simulink model "gm_PMLSM_FOC_FixedPoint"  (R2026b)
settings: Solver=FixedStepDiscrete  StopTime=0.0063  FixedStep=2e-08
undefined symbols (not defined in the file): Lookup, Ts_ACR
libraries: hdlmdlgenlib x38, simulink x8
(part 1 of 5)
settings Model: Creator=lww  LastModifiedBy=lww
settings DataIOCC: ExternalInput=M3_HDL_Stimulus  LoadExternalInput=on
settings OptimizationCC: BlockReduction=off  ConditionallyExecuteInputs=off  DefaultParameterBehavior=Inlined
settings DebuggingCC: FixptConstOverflowMsg=error  InheritedTsInSrcMsg=none  IntegerOverflowMsg=error  IntegerSaturationMsg=error

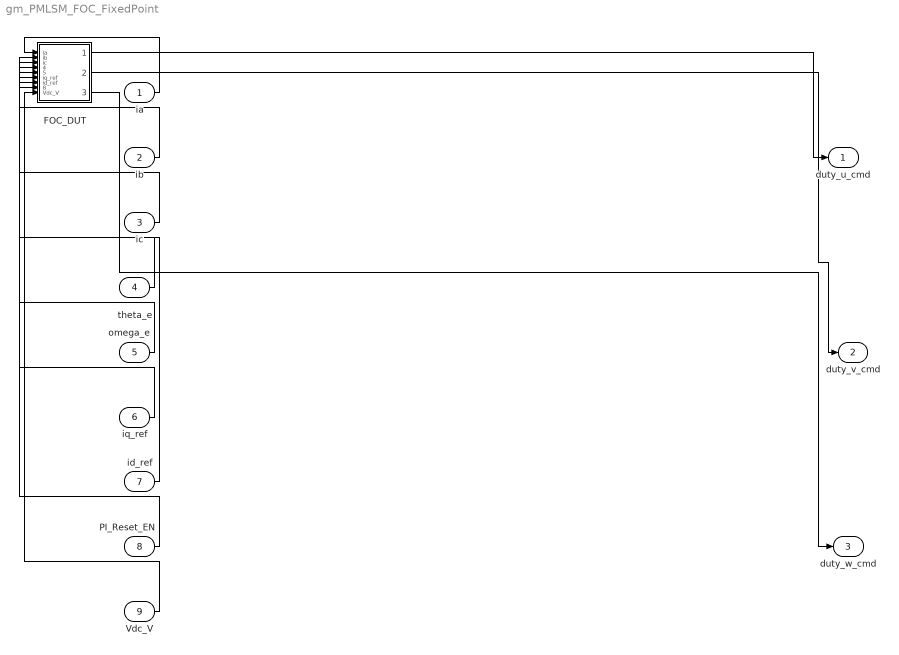
== system gm_PMLSM_FOC_FixedPoint ==
  ia : Inport  OutDataTypeStr=FOC_Fixed_Config.Types.Current  SampleTime=Ts_ACR  Interpolate=off
  ib : Inport  Port=2  OutDataTypeStr=FOC_Fixed_Config.Types.Current  SampleTime=Ts_ACR  Interpolate=off
  ic : Inport  Port=3  OutDataTypeStr=FOC_Fixed_Config.Types.Current  SampleTime=Ts_ACR  Interpolate=off
  theta_e : Inport  Port=4  OutDataTypeStr=FOC_Fixed_Config.Types.Angle  SampleTime=Ts_ACR  Interpolate=off
  omega_e : Inport  Port=5  OutDataTypeStr=FOC_Fixed_Config.Types.Omega  SampleTime=Ts_ACR  Interpolate=off
  iq_ref : Inport  Port=6  OutDataTypeStr=FOC_Fixed_Config.Types.Current  SampleTime=Ts_ACR  Interpolate=off
  id_ref : Inport  Port=7  OutDataTypeStr=FOC_Fixed_Config.Types.Current  SampleTime=Ts_ACR  Interpolate=off
  PI_Reset_EN : Inport  Port=8  OutDataTypeStr=boolean  SampleTime=Ts_ACR  Interpolate=off
  Vdc_V : Inport  Port=9  OutDataTypeStr=FOC_Fixed_Config.Types.Bus  SampleTime=Ts_ACR  Interpolate=off
  FOC_DUT : Subsystem
  duty_u_cmd : Outport  OutDataTypeStr=FOC_Fixed_Config.Types.Duty
  duty_v_cmd : Outport  Port=2  OutDataTypeStr=FOC_Fixed_Config.Types.Duty
  duty_w_cmd : Outport  Port=3  OutDataTypeStr=FOC_Fixed_Config.Types.Duty
  wires:
  Vdc_V/1 -> FOC_DUT/9(Vdc_V)
  FOC_DUT/3(duty_w_cmd) -> duty_w_cmd/1
  FOC_DUT/2(duty_v_cmd) -> duty_v_cmd/1
  FOC_DUT/1(duty_u_cmd) -> duty_u_cmd/1
  PI_Reset_EN/1 -> FOC_DUT/8(PI_Reset_EN)
  id_ref/1 -> FOC_DUT/7(id_ref)
  iq_ref/1 -> FOC_DUT/6(iq_ref)
  omega_e/1 -> FOC_DUT/5(omega_e)
  theta_e/1 -> FOC_DUT/4(theta_e)
  ic/1 -> FOC_DUT/3(ic)
  ib/1 -> FOC_DUT/2(ib)
  ia/1 -> FOC_DUT/1(ia)

== system gm_PMLSM_FOC_FixedPoint/FOC_DUT ==
  ia : Inport  OutDataTypeStr=fixdt(1, 32, 24)  PortDimensions=1  SampleTime=0.0001
  ib : Inport  Port=2  OutDataTypeStr=fixdt(1, 32, 24)  PortDimensions=1  SampleTime=0.0001
  ic : Inport  Port=3  OutDataTypeStr=fixdt(1, 32, 24)  PortDimensions=1  SampleTime=0.0001
  theta_e : Inport  Port=4  OutDataTypeStr=fixdt(1, 40, 32)  PortDimensions=1  SampleTime=0.0001
  omega_e : Inport  Port=5  OutDataTypeStr=fixdt(1, 40, 24)  PortDimensions=1  SampleTime=0.0001
  iq_ref : Inport  Port=6  OutDataTypeStr=fixdt(1, 32, 24)  PortDimensions=1  SampleTime=0.0001
  id_ref : Inport  Port=7  OutDataTypeStr=fixdt(1, 32, 24)  PortDimensions=1  SampleTime=0.0001
  PI_Reset_EN : Inport  Port=8  OutDataTypeStr=boolean  PortDimensions=1  SampleTime=0.0001
  Vdc_V : Inport  Port=9  OutDataTypeStr=fixdt(0, 32, 24)  PortDimensions=1  SampleTime=0.0001
  FOC_DUT : Subsystem  TreatAsAtomicUnit=on
  t : RateTransition  OutPortSampleTimeOpt=Multiple of input port sample time  OutPortSampleTimeMultiple=5000
  t1 : RateTransition  OutPortSampleTimeOpt=Multiple of input port sample time  OutPortSampleTimeMultiple=5000
  t2 : RateTransition  OutPortSampleTimeOpt=Multiple of input port sample time  OutPortSampleTimeMultiple=5000
  duty_u_cmd : Outport  OutDataTypeStr=fixdt(0, 32, 30)  PortDimensions=1  SampleTime=0.0001
  duty_v_cmd : Outport  Port=2  OutDataTypeStr=fixdt(0, 32, 30)  PortDimensions=1  SampleTime=0.0001
  duty_w_cmd : Outport  Port=3  OutDataTypeStr=fixdt(0, 32, 30)  PortDimensions=1  SampleTime=0.0001
  wires:
  id_ref/1 -> FOC_DUT/7(id_ref)
  iq_ref/1 -> FOC_DUT/6(iq_ref)
  omega_e/1 -> FOC_DUT/5(omega_e)
  theta_e/1 -> FOC_DUT/4(theta_e)
  ic/1 -> FOC_DUT/3(ic)
  ia/1 -> FOC_DUT/1(ia)
  ib/1 -> FOC_DUT/2(ib)
  PI_Reset_EN/1 -> FOC_DUT/8(PI_Reset_EN)
  FOC_DUT/2(duty_v_cmd) -> t1/1
  Vdc_V/1 -> FOC_DUT/9(Vdc_V)
  FOC_DUT/1(duty_u_cmd) -> t/1
  FOC_DUT/3(duty_w_cmd) -> t2/1
  t/1 -> duty_u_cmd/1
  t1/1 -> duty_v_cmd/1
  t2/1 -> duty_w_cmd/1

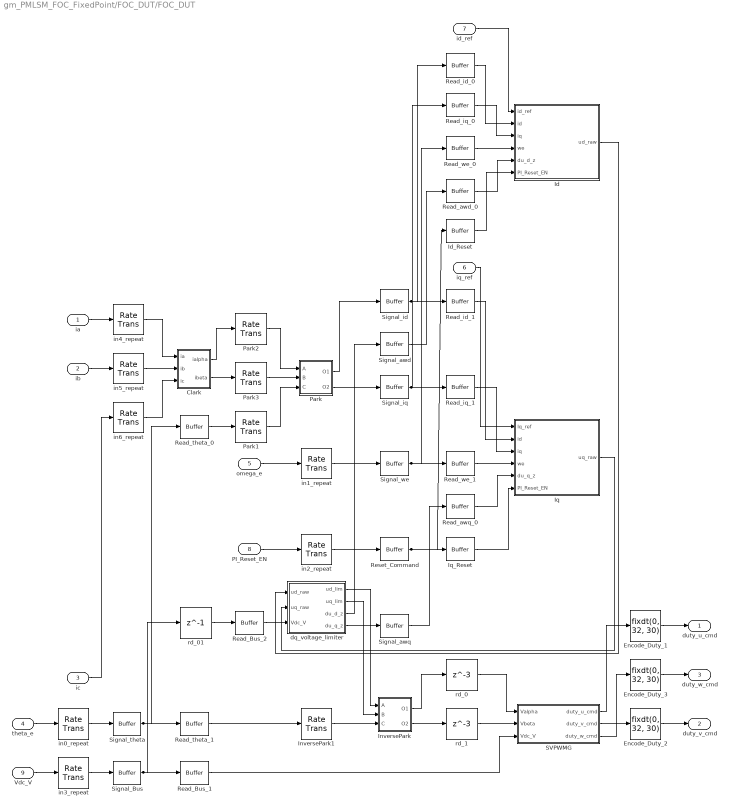
== system gm_PMLSM_FOC_FixedPoint/FOC_DUT/FOC_DUT ==
  ia : Inport  OutDataTypeStr=fixdt(1,32,24,'DataTypeOverride', 'Off')  PortDimensions=1  SampleTime=0.0001
  ib : Inport  Port=2  OutDataTypeStr=fixdt(1,32,24,'DataTypeOverride', 'Off')  PortDimensions=1  SampleTime=0.0001
  ic : Inport  Port=3  OutDataTypeStr=fixdt(1,32,24,'DataTypeOverride', 'Off')  PortDimensions=1  SampleTime=0.0001
  theta_e : Inport  Port=4  OutDataTypeStr=fixdt(1,40,32,'DataTypeOverride', 'Off')  PortDimensions=1  SampleTime=0.0001
  omega_e : Inport  Port=5  OutDataTypeStr=fixdt(1,40,24,'DataTypeOverride', 'Off')  PortDimensions=1  SampleTime=0.0001
  iq_ref : Inport  Port=6  OutDataTypeStr=fixdt(1,32,24,'DataTypeOverride', 'Off')  PortDimensions=1  SampleTime=0.0001
  id_ref : Inport  Port=7  OutDataTypeStr=fixdt(1,32,24,'DataTypeOverride', 'Off')  PortDimensions=1  SampleTime=0.0001
  PI_Reset_EN : Inport  Port=8  OutDataTypeStr=boolean  PortDimensions=1  SampleTime=0.0001
  Vdc_V : Inport  Port=9  OutDataTypeStr=fixdt(0,32,24,'DataTypeOverride', 'Off')  PortDimensions=1  SampleTime=0.0001
  Clark : Subsystem
  Encode_Duty_1 : DataTypeConversion  OutDataTypeStr=fixdt(0, 32, 30)  RndMeth=Convergent  SampleTime=2e-08
  Encode_Duty_2 : DataTypeConversion  OutDataTypeStr=fixdt(0, 32, 30)  RndMeth=Convergent  SampleTime=2e-08
  Encode_Duty_3 : DataTypeConversion  OutDataTypeStr=fixdt(0, 32, 30)  RndMeth=Convergent  SampleTime=2e-08
  Id : Subsystem
  Id_Reset : hdlmdlgenlib/Buffer
  InversePark : Subsystem  mask(Park to Clarke Angle Transform){AxisAlignment=D-axis, UseWithEmbedded=on, PhaseInput='Two inputs', ThetaInput=Electrical position, AngleInput=Radians, N_points=1024}
      mask prompts: AxisAlignment "shared_mcbeeblks:mcbeeblks:InvPBlkPrmAlign"; UseWithEmbedded "shared_mcbeeblks:mcbeeblks:BlkEmbeddedUse"; PhaseInput "shared_mcbeeblks:mcbeeblks:InvPPrmInp"; ThetaInput "shared_mcbeeblks:mcbeeblks:InvPPrmTheta"; AngleInput "shared_mcbeeblks:mcbeeblks:InvPThetaUnits"; N_points "shared_mcbeeblks:mcbeeblks:InvPPrmLUTSize"
      mask help: shared_mcbeeblks:mcbeeblks:InvPBlkDlgDes
      mask init:
      | AngleInput = 2;
      | AxisAlignment = 1;
      | N_points = 1024;
      | PhaseInput = 1;
      | ThetaInput = 1;
      | UseWithEmbedded = 1;
      mask Help: eval('mcbeeutil.mcbeesharedhelp(''inverseparktransform'')')
      mask TypeOptions AxisAlignment: shared_mcbeeblks:mcbeeblks:InvPpopDaxis | shared_mcbeeblks:mcbeeblks:InvPpopQaxis
      mask Callback UseWithEmbedded: mcbeeutil.mcbeeParkToClarkeCb('embeddeduse',gcbh);
      mask TypeOptions ThetaInput: shared_mcbeeblks:mcbeeblks:InvPPopElec | shared_mcbeeblks:mcbeeblks:InvPPopSinCos
      mask Callback ThetaInput: mcbeeutil.mcbeeParkToClarkeCb('ThetaInputCb',gcbh);
      mask TypeOptions AngleInput: shared_mcbeeblks:mcbeeblks:InvPPopPUUnit | shared_mcbeeblks:mcbeeblks:InvPPopRadUnit | shared_mcbeeblks:mcbeeblks:InvPPopDegUnit
      mask Display:
      | fprintf('Park to\nClarke')
      | port_label('input',1, 'd','interpreter', 'tex');
      | port_label('input',2, 'q','interpreter', 'tex');
      | port_label('input',3, '\theta_e','interpreter', 'tex');
      | port_label('output',1, '\alpha','interpreter', 'tex');
      | port_label('output',2, '\beta','interpreter', 'tex');
  InversePark1 : RateTransition  OutPortSampleTimeOpt=Multiple of input port sample time  OutPortSampleTimeMultiple=5000
  Iq : Subsystem
  Iq_Reset : hdlmdlgenlib/Buffer
  Park : Subsystem  mask(Clarke to Park Angle Transform){AxisAlignment=D-axis, UseWithEmbedded=on, PhaseInput='Two inputs', ThetaInput=Electrical position, AngleInput=Radians, N_points=1024}
      mask prompts: AxisAlignment "shared_mcbeeblks:mcbeeblks:ParkBlkPrmAlign"; UseWithEmbedded "shared_mcbeeblks:mcbeeblks:BlkEmbeddedUse"; PhaseInput "shared_mcbeeblks:mcbeeblks:ParkPrmInp"; ThetaInput "shared_mcbeeblks:mcbeeblks:ParkPrmTheta"; AngleInput "shared_mcbeeblks:mcbeeblks:ParkPrmThetaUnits"; N_points "shared_mcbeeblks:mcbeeblks:ParkPrmLUTSize"
      mask help: shared_mcbeeblks:mcbeeblks:ParkBlkDlgDes
      mask init:
      | AngleInput = 2;
      | AxisAlignment = 1;
      | N_points = 1024;
      | PhaseInput = 1;
      | ThetaInput = 1;
      | UseWithEmbedded = 1;
      mask Help: eval('mcbeeutil.mcbeesharedhelp(''parktransform'')')
      mask TypeOptions AxisAlignment: shared_mcbeeblks:mcbeeblks:ParkpopDaxis | shared_mcbeeblks:mcbeeblks:ParkpopQaxis
      mask Callback UseWithEmbedded: mcbeeutil.mcbeeClarkeToParkCb('embeddeduse',gcbh);
      mask TypeOptions ThetaInput: shared_mcbeeblks:mcbeeblks:ParkPopElec | shared_mcbeeblks:mcbeeblks:ParkPopSinCos
      mask Callback ThetaInput: mcbeeutil.mcbeeClarkeToParkCb('ThetaInputCb',gcbh)
      mask TypeOptions AngleInput: shared_mcbeeblks:mcbeeblks:ParkPopPUUnit | shared_mcbeeblks:mcbeeblks:ParkPopRadUnit | shared_mcbeeblks:mcbeeblks:ParkPopDegUnit
      mask Display:
      | fprintf('Clarke to\nPark')
      | port_label('input',1, '\alpha','interpreter', 'tex');
      | port_label('input',2, '\beta','interpreter', 'tex');
      | port_label('input',3, '\theta_e','interpreter', 'tex');
      | port_label('output',1, 'd','interpreter', 'tex');
      | port_label('output',2, 'q','interpreter', 'tex');
  Park1 : RateTransition  OutPortSampleTimeOpt=Multiple of input port sample time  OutPortSampleTimeMultiple=5000
  Park2 : RateTransition  OutPortSampleTimeOpt=Multiple of input port sample time  OutPortSampleTimeMultiple=5000
  Park3 : RateTransition  OutPortSampleTimeOpt=Multiple of input port sample time  OutPortSampleTimeMultiple=5000
  Read_Bus_1 : hdlmdlgenlib/Buffer
  Read_Bus_2 : hdlmdlgenlib/Buffer
  Read_awd_0 : hdlmdlgenlib/Buffer
  Read_awq_0 : hdlmdlgenlib/Buffer
  Read_id_0 : hdlmdlgenlib/Buffer
  Read_id_1 : hdlmdlgenlib/Buffer
  Read_iq_0 : hdlmdlgenlib/Buffer
  Read_iq_1 : hdlmdlgenlib/Buffer
  Read_theta_0 : hdlmdlgenlib/Buffer
  Read_theta_1 : hdlmdlgenlib/Buffer
  Read_we_0 : hdlmdlgenlib/Buffer
  Read_we_1 : hdlmdlgenlib/Buffer
  Reset_Command : hdlmdlgenlib/Buffer
  SVPWMG : Subsystem
  Signal_Bus : hdlmdlgenlib/Buffer
  Signal_awd : hdlmdlgenlib/Buffer
  Signal_awq : hdlmdlgenlib/Buffer
  Signal_id : hdlmdlgenlib/Buffer
  Signal_iq : hdlmdlgenlib/Buffer
  Signal_theta : hdlmdlgenlib/Buffer
  Signal_we : hdlmdlgenlib/Buffer
  dq_voltage_limiter : Subsystem
  in0_repeat : RateTransition  Integrity=off  Deterministic=off  OutPortSampleTimeOpt=Multiple of input port sample time  OutPortSampleTimeMultiple=1/5000
  in1_repeat : RateTransition  Integrity=off  Deterministic=off  OutPortSampleTimeOpt=Multiple of input port sample time  OutPortSampleTimeMultiple=1/5000
  in2_repeat : RateTransition  Integrity=off  Deterministic=off  OutPortSampleTimeOpt=Multiple of input port sample time  OutPortSampleTimeMultiple=1/5000
  in3_repeat : RateTransition  Integrity=off  Deterministic=off  OutPortSampleTimeOpt=Multiple of input port sample time  OutPortSampleTimeMultiple=1/5000
  in4_repeat : RateTransition  Integrity=off  Deterministic=off  OutPortSampleTimeOpt=Multiple of input port sample time  OutPortSampleTimeMultiple=1/5000
  in5_repeat : RateTransition  Integrity=off  Deterministic=off  OutPortSampleTimeOpt=Multiple of input port sample time  OutPortSampleTimeMultiple=1/5000
  in6_repeat : RateTransition  Integrity=off  Deterministic=off  OutPortSampleTimeOpt=Multiple of input port sample time  OutPortSampleTimeMultiple=1/5000
  rd_0 : Delay  DelayLength=3  InitialCondition=0  SampleTime=2e-08
  rd_01 : Delay  DelayLength=1  InitialCondition=0  SampleTime=2e-08
  rd_1 : Delay  DelayLength=3  InitialCondition=0  SampleTime=2e-08
  duty_u_cmd : Outport  OutDataTypeStr=fixdt(0,32,30,'DataTypeOverride', 'Off')  PortDimensions=1  SampleTime=2e-08
  duty_v_cmd : Outport  Port=2  OutDataTypeStr=fixdt(0,32,30,'DataTypeOverride', 'Off')  PortDimensions=1  SampleTime=2e-08
  duty_w_cmd : Outport  Port=3  OutDataTypeStr=fixdt(0,32,30,'DataTypeOverride', 'Off')  PortDimensions=1  SampleTime=2e-08
  wires:
  Signal_id/1 -> Read_id_1/1, Read_id_0/1
  theta_e/1 -> in0_repeat/1
  ia/1 -> in4_repeat/1
  Vdc_V/1 -> in3_repeat/1
  in3_repeat/1 -> Signal_Bus/1
  ib/1 -> in5_repeat/1
  SVPWMG/3(duty_w_cmd) -> Encode_Duty_3/1
  Signal_Bus/1 -> Read_Bus_1/1, rd_01/1
  ic/1 -> in6_repeat/1
  Read_awd_0/1 -> Id/5(du_d_z)
  in0_repeat/1 -> Signal_theta/1
  dq_voltage_limiter/2(uq_lim) -> InversePark/2(B)
  in4_repeat/1 -> Clark/1(ia)
  in5_repeat/1 -> Clark/2(ib)
  rd_1/1 -> SVPWMG/2(Vbeta)
  Reset_Command/1 -> Iq_Reset/1, Id_Reset/1
  in6_repeat/1 -> Clark/3(ic)
  Signal_theta/1 -> Read_theta_0/1, Read_theta_1/1
  Clark/1(ialpha) -> Park2/1
  Read_id_0/1 -> Id/2(id)
  Clark/2(ibeta) -> Park3/1
  InversePark/2(O2) -> rd_1/1
  Read_theta_0/1 -> Park1/1
  Encode_Duty_2/1 -> duty_v_cmd/1
  Signal_awq/1 -> Read_awq_0/1
  rd_01/1 -> Read_Bus_2/1
  Read_theta_1/1 -> InversePark1/1
  Read_Bus_1/1 -> SVPWMG/3(Vdc_V)
  Id/1(ud_raw) -> dq_voltage_limiter/1(ud_raw)
  Iq_Reset/1 -> Iq/6(PI_Reset_EN)
  Park2/1 -> Park/1(A)
  Park3/1 -> Park/2(B)
  Park1/1 -> Park/3(C)
  omega_e/1 -> in1_repeat/1
  PI_Reset_EN/1 -> in2_repeat/1
  id_ref/1 -> Id/1(id_ref)
  Read_Bus_2/1 -> dq_voltage_limiter/3(Vdc_V)
  Park/1(O1) -> Signal_id/1
  SVPWMG/2(duty_v_cmd) -> Encode_Duty_2/1
  Park/2(O2) -> Signal_iq/1
  Id_Reset/1 -> Id/6(PI_Reset_EN)
  in1_repeat/1 -> Signal_we/1
  in2_repeat/1 -> Reset_Command/1
  Encode_Duty_1/1 -> duty_u_cmd/1
  dq_voltage_limiter/1(ud_lim) -> InversePark/1(A)
  Read_we_1/1 -> Iq/4(we)
  dq_voltage_limiter/3(du_d_z) -> Signal_awd/1
  SVPWMG/1(duty_u_cmd) -> Encode_Duty_1/1
  dq_voltage_limiter/4(du_q_z) -> Signal_awq/1
  InversePark1/1 -> InversePark/3(C)
  Signal_awd/1 -> Read_awd_0/1
  Signal_iq/1 -> Read_iq_1/1, Read_iq_0/1
  Signal_we/1 -> Read_we_1/1, Read_we_0/1
  InversePark/1(O1) -> rd_0/1
  Read_iq_0/1 -> Id/3(iq)
  Read_we_0/1 -> Id/4(we)
  iq_ref/1 -> Iq/1(Iq_ref)
  rd_0/1 -> SVPWMG/1(Valpha)
  Read_id_1/1 -> Iq/2(id)
  Read_iq_1/1 -> Iq/3(iq)
  Read_awq_0/1 -> Iq/5(du_q_z)
  Iq/1(uq_raw) -> dq_voltage_limiter/2(uq_raw)
  Encode_Duty_3/1 -> duty_w_cmd/1

== system gm_PMLSM_FOC_FixedPoint/FOC_DUT/FOC_DUT/Clark ==
  ia : Inport  OutDataTypeStr=fixdt(1, 32, 24)  PortDimensions=1  SampleTime=2e-08
  ib : Inport  Port=2  OutDataTypeStr=fixdt(1, 32, 24)  PortDimensions=1  SampleTime=2e-08
  ic : Inport  Port=3  OutDataTypeStr=fixdt(1, 32, 24)  PortDimensions=1  SampleTime=2e-08
  Add1 : Sum  Inputs=+-  OutDataTypeStr=fixdt(1, 64, 40)  AccumDataTypeStr=fixdt(1, 64, 40)  RndMeth=Convergent  SaturateOnIntegerOverflow=on  SampleTime=2e-08
  Add_stage2 : Sum  Inputs=+-  OutDataTypeStr=fixdt(1, 64, 40)  AccumDataTypeStr=fixdt(1, 64, 40)  RndMeth=Convergent  SaturateOnIntegerOverflow=on  SampleTime=2e-08
  Add_stage3 : Sum  Inputs=+-  OutDataTypeStr=fixdt(1, 64, 40)  AccumDataTypeStr=fixdt(1, 64, 40)  RndMeth=Convergent  SaturateOnIntegerOverflow=on  SampleTime=2e-08
  Gain : Gain  Gain="fi(0,1,64,40,\"hex\",\"0000008000000000\")"  ParamDataTypeStr=fixdt(1, 64, 40)  OutDataTypeStr=fixdt(1, 64, 40)  RndMeth=Convergent  SaturateOnIntegerOverflow=on  SampleTime=2e-08
  Gain1 : Gain  Gain="fi(0,1,64,40,\"hex\",\"0000008000000000\")"  ParamDataTypeStr=fixdt(1, 64, 40)  OutDataTypeStr=fixdt(1, 64, 40)  RndMeth=Convergent  SaturateOnIntegerOverflow=on  SampleTime=2e-08
  Gain2 : Gain  Gain="fi(0,1,64,40,\"hex\",\"000000aaaaaaaaab\")"  ParamDataTypeStr=fixdt(1, 64, 40)  OutDataTypeStr=fixdt(1, 128, 80)  SampleTime=2e-08
  Gain2_out_dtc : DataTypeConversion  OutDataTypeStr=fixdt(1, 64, 40)  RndMeth=Convergent  SampleTime=2e-08
  Gain3 : Gain  Gain="fi(0,1,64,40,\"hex\",\"00000093cd3a2c82\")"  ParamDataTypeStr=fixdt(1, 64, 40)  OutDataTypeStr=fixdt(1, 128, 80)  SampleTime=2e-08
  Gain3_out_dtc : DataTypeConversion  OutDataTypeStr=fixdt(1, 64, 40)  RndMeth=Convergent  SampleTime=2e-08
  ialpha : Outport  OutDataTypeStr=fixdt(1, 64, 40)  PortDimensions=1  SampleTime=2e-08
  ibeta : Outport  Port=2  OutDataTypeStr=fixdt(1, 64, 40)  PortDimensions=1  SampleTime=2e-08
  wires:
  Gain1/1 -> Add_stage3/2
  ib/1 -> Add1/1, Gain/1
  Add1/1 -> Gain3/1
  ic/1 -> Gain1/1, Add1/2
  Gain/1 -> Add_stage2/2
  ia/1 -> Add_stage2/1
  Add_stage2/1 -> Add_stage3/1
  Gain3/1 -> Gain3_out_dtc/1
  Add_stage3/1 -> Gain2/1
  Gain3_out_dtc/1 -> ibeta/1
  Gain2/1 -> Gain2_out_dtc/1
  Gain2_out_dtc/1 -> ialpha/1

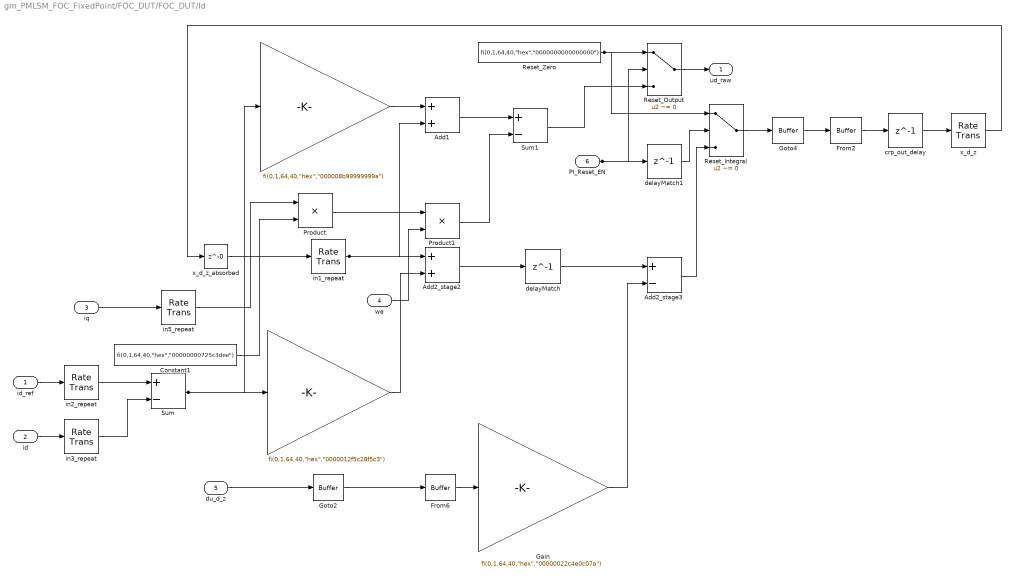
== system gm_PMLSM_FOC_FixedPoint/FOC_DUT/FOC_DUT/Id ==
  id_ref : Inport  OutDataTypeStr=fixdt(1, 32, 24)  PortDimensions=1  SampleTime=0.0001
  id : Inport  Port=2  OutDataTypeStr=fixdt(1, 64, 40)  PortDimensions=1  SampleTime=0.0001
  iq : Inport  Port=3  OutDataTypeStr=fixdt(1, 64, 40)  PortDimensions=1  SampleTime=0.0001
  we : Inport  Port=4  OutDataTypeStr=fixdt(1, 40, 24)  PortDimensions=1  SampleTime=2e-08
  du_d_z : Inport  Port=5  OutDataTypeStr=fixdt(1, 64, 40)  PortDimensions=1  SampleTime=2e-08
  PI_Reset_EN : Inport  Port=6  OutDataTypeStr=boolean  PortDimensions=1  SampleTime=2e-08
  " " : Gain  Gain="fi(0,1,64,40,\"hex\",\"0000012f5c28f5c3\")"  ParamDataTypeStr=fixdt(1, 64, 40)  OutDataTypeStr=fixdt(1, 64, 40)  RndMeth=Convergent  SaturateOnIntegerOverflow=on  SampleTime=2e-08
  "  " : Gain  Gain="fi(0,1,64,40,\"hex\",\"000008b99999999a\")"  ParamDataTypeStr=fixdt(1, 64, 40)  OutDataTypeStr=fixdt(1, 64, 40)  RndMeth=Convergent  SaturateOnIntegerOverflow=on  SampleTime=2e-08
  Add1 : Sum  OutDataTypeStr=fixdt(1, 64, 40)  AccumDataTypeStr=fixdt(1, 64, 40)  RndMeth=Convergent  SaturateOnIntegerOverflow=on  SampleTime=2e-08
  Add2_stage2 : Sum  OutDataTypeStr=fixdt(1, 64, 40)  AccumDataTypeStr=fixdt(1, 64, 40)  RndMeth=Convergent  SaturateOnIntegerOverflow=on  SampleTime=2e-08
  Add2_stage3 : Sum  Inputs=+-  OutDataTypeStr=fixdt(1, 64, 40)  AccumDataTypeStr=fixdt(1, 64, 40)  RndMeth=Convergent  SaturateOnIntegerOverflow=on  SampleTime=2e-08
  Constant1 : Constant  Value="fi(0,1,64,40,\"hex\",\"00000000725c3dee\")"  OutDataTypeStr=fixdt(1, 64, 40)  SampleTime=2e-08
  From2 : hdlmdlgenlib/Buffer
  From6 : hdlmdlgenlib/Buffer
  Gain : Gain  Gain="fi(0,1,64,40,\"hex\",\"00000022c4e0c07a\")"  ParamDataTypeStr=fixdt(1, 64, 40)  OutDataTypeStr=fixdt(1, 64, 40)  RndMeth=Convergent  SaturateOnIntegerOverflow=on  SampleTime=2e-08
  Goto2 : hdlmdlgenlib/Buffer
  Goto4 : hdlmdlgenlib/Buffer
  Product : Product  Inputs=**  OutDataTypeStr=fixdt(1, 64, 40)  RndMeth=Convergent  SaturateOnIntegerOverflow=on  SampleTime=2e-08
  Product1 : Product  Inputs=**  OutDataTypeStr=fixdt(1, 64, 40)  RndMeth=Convergent  SaturateOnIntegerOverflow=on  SampleTime=2e-08
  Reset_Integral : Switch  Criteria=u2 ~= 0  Threshold="fi(0,0,1,0,\"hex\",\"0\")"  OutDataTypeStr=fixdt(1, 64, 40)  RndMeth=Convergent  SampleTime=2e-08  InputSameDT=off
  Reset_Output : Switch  Criteria=u2 ~= 0  Threshold="fi(0,0,1,0,\"hex\",\"0\")"  OutDataTypeStr=fixdt(1, 64, 40)  RndMeth=Convergent  SampleTime=2e-08  InputSameDT=off
  Reset_Zero : Constant  Value="fi(0,1,64,40,\"hex\",\"0000000000000000\")"  OutDataTypeStr=fixdt(1, 64, 40)  SampleTime=2e-08
  Sum : Sum  Inputs=+-  OutDataTypeStr=fixdt(1, 64, 40)  AccumDataTypeStr=fixdt(1, 64, 40)  RndMeth=Convergent  SaturateOnIntegerOverflow=on  SampleTime=2e-08
  Sum1 : Sum  Inputs=+-  OutDataTypeStr=fixdt(1, 64, 40)  AccumDataTypeStr=fixdt(1, 64, 40)  RndMeth=Convergent  SaturateOnIntegerOverflow=on  SampleTime=2e-08
  crp_out_delay : Delay  DelayLength=1  InitialCondition=0  SampleTime=2e-08
  delayMatch : Delay  DelayLength=1  InitialCondition=0  SampleTime=2e-08
  delayMatch1 : Delay  DelayLength=1  InitialCondition=0  SampleTime=2e-08
  in1_repeat : RateTransition  Integrity=off  Deterministic=off  OutPortSampleTimeOpt=Multiple of input port sample time  OutPortSampleTimeMultiple=1/5000
  in2_repeat : RateTransition  Integrity=off  Deterministic=off  OutPortSampleTimeOpt=Multiple of input port sample time  OutPortSampleTimeMultiple=1/5000
  in3_repeat : RateTransition  Integrity=off  Deterministic=off  OutPortSampleTimeOpt=Multiple of input port sample time  OutPortSampleTimeMultiple=1/5000
  in5_repeat : RateTransition  Integrity=off  Deterministic=off  OutPortSampleTimeOpt=Multiple of input port sample time  OutPortSampleTimeMultiple=1/5000
  x_d_z : RateTransition  OutPortSampleTimeOpt=Multiple of input port sample time  OutPortSampleTimeMultiple=5000
  x_d_z_absorbed : Delay  DelayLength=0
  ud_raw : Outport  OutDataTypeStr=fixdt(1, 64, 40)  PortDimensions=1  SampleTime=2e-08
  wires:
  From6/1 -> Gain/1
  Goto2/1 -> From6/1
  in5_repeat/1 -> Product/1
  id_ref/1 -> in2_repeat/1
  x_d_z_absorbed/1 -> in1_repeat/1
  id/1 -> in3_repeat/1
  in3_repeat/1 -> Sum/2
  iq/1 -> in5_repeat/1
  in2_repeat/1 -> Sum/1
  Constant1/1 -> Product/2
  we/1 -> Product1/2
  Sum/1 -> "  "/1, " "/1
  Product1/1 -> Sum1/2
  du_d_z/1 -> Goto2/1
  "  "/1 -> Add1/1
  Product/1 -> Product1/1
  in1_repeat/1 -> Add1/2, Add2_stage2/1
  " "/1 -> Add2_stage2/2
  Add1/1 -> Sum1/1
  Add2_stage2/1 -> delayMatch/1
  PI_Reset_EN/1 -> delayMatch1/1, Reset_Output/2
  Reset_Zero/1 -> Reset_Integral/1, Reset_Output/1
  Sum1/1 -> Reset_Output/3
  delayMatch/1 -> Add2_stage3/1
  x_d_z/1 -> x_d_z_absorbed/1
  Gain/1 -> Add2_stage3/2
  Reset_Output/1 -> ud_raw/1
  delayMatch1/1 -> Reset_Integral/2
  Add2_stage3/1 -> Reset_Integral/3
  Reset_Integral/1 -> Goto4/1
  Goto4/1 -> From2/1
  From2/1 -> crp_out_delay/1
  crp_out_delay/1 -> x_d_z/1

== system gm_PMLSM_FOC_FixedPoint/FOC_DUT/FOC_DUT/InversePark ==
  A : Inport  OutDataTypeStr=fixdt(1,64,40,'DataTypeOverride', 'Off')  PortDimensions=1  SampleTime=2e-08
  B : Inport  Port=2  OutDataTypeStr=fixdt(1,64,40,'DataTypeOverride', 'Off')  PortDimensions=1  SampleTime=2e-08
  C : Inport  Port=3  OutDataTypeStr=fixdt(1,40,32,'DataTypeOverride', 'Off')  PortDimensions=1  SampleTime=0.0001
  Variant : Subsystem
  O1 : Outport  OutDataTypeStr=fixdt(1, 64, 40)  PortDimensions=1  SampleTime=2e-08
  O2 : Outport  Port=2  OutDataTypeStr=fixdt(1, 64, 40)  PortDimensions=1  SampleTime=2e-08
  wires:
  A/1 -> Variant/1(A)
  B/1 -> Variant/2(B)
  C/1 -> Variant/3(C)
  Variant/1(O1) -> O1/1
  Variant/2(O2) -> O2/1

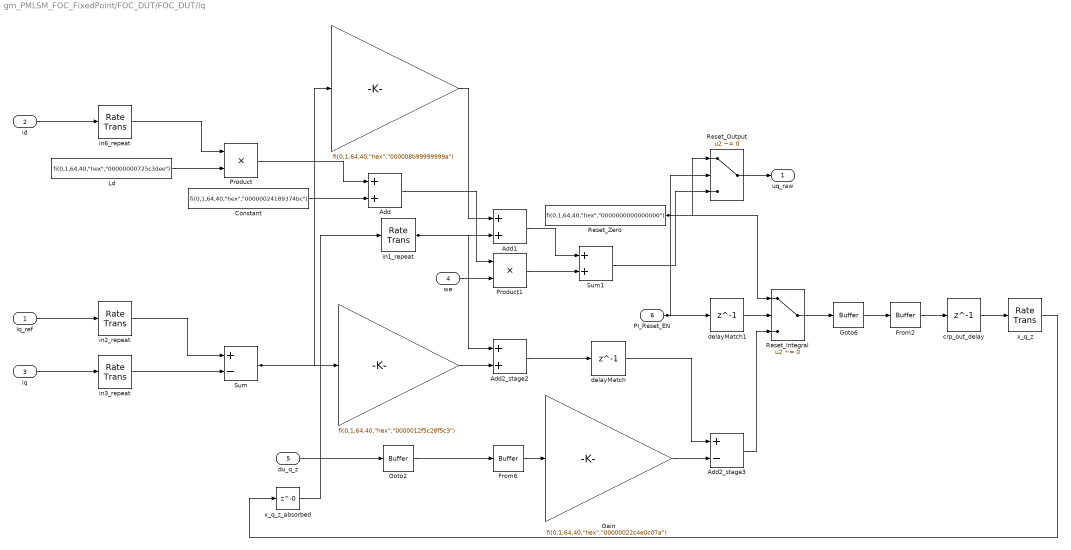
== system gm_PMLSM_FOC_FixedPoint/FOC_DUT/FOC_DUT/Iq ==
  Iq_ref : Inport  OutDataTypeStr=fixdt(1, 32, 24)  PortDimensions=1  SampleTime=0.0001
  id : Inport  Port=2  OutDataTypeStr=fixdt(1, 64, 40)  PortDimensions=1  SampleTime=0.0001
  iq : Inport  Port=3  OutDataTypeStr=fixdt(1, 64, 40)  PortDimensions=1  SampleTime=0.0001
  we : Inport  Port=4  OutDataTypeStr=fixdt(1, 40, 24)  PortDimensions=1  SampleTime=2e-08
  du_q_z : Inport  Port=5  OutDataTypeStr=fixdt(1, 64, 40)  PortDimensions=1  SampleTime=2e-08
  PI_Reset_EN : Inport  Port=6  OutDataTypeStr=boolean  PortDimensions=1  SampleTime=2e-08
  " " : Gain  Gain="fi(0,1,64,40,\"hex\",\"0000012f5c28f5c3\")"  ParamDataTypeStr=fixdt(1, 64, 40)  OutDataTypeStr=fixdt(1, 64, 40)  RndMeth=Convergent  SaturateOnIntegerOverflow=on  SampleTime=2e-08
  "  " : Gain  Gain="fi(0,1,64,40,\"hex\",\"000008b99999999a\")"  ParamDataTypeStr=fixdt(1, 64, 40)  OutDataTypeStr=fixdt(1, 64, 40)  RndMeth=Convergent  SaturateOnIntegerOverflow=on  SampleTime=2e-08
  Add : Sum  OutDataTypeStr=fixdt(1, 64, 40)  AccumDataTypeStr=fixdt(1, 64, 40)  RndMeth=Convergent  SaturateOnIntegerOverflow=on  SampleTime=2e-08
  Add1 : Sum  OutDataTypeStr=fixdt(1, 64, 40)  AccumDataTypeStr=fixdt(1, 64, 40)  RndMeth=Convergent  SaturateOnIntegerOverflow=on  SampleTime=2e-08
  Add2_stage2 : Sum  OutDataTypeStr=fixdt(1, 64, 40)  AccumDataTypeStr=fixdt(1, 64, 40)  RndMeth=Convergent  SaturateOnIntegerOverflow=on  SampleTime=2e-08
  Add2_stage3 : Sum  Inputs=+-  OutDataTypeStr=fixdt(1, 64, 40)  AccumDataTypeStr=fixdt(1, 64, 40)  RndMeth=Convergent  SaturateOnIntegerOverflow=on  SampleTime=2e-08
  Constant : Constant  Value="fi(0,1,64,40,\"hex\",\"00000024189374bc\")"  OutDataTypeStr=fixdt(1, 64, 40)  SampleTime=2e-08
  From2 : hdlmdlgenlib/Buffer
  From6 : hdlmdlgenlib/Buffer
  Gain : Gain  Gain="fi(0,1,64,40,\"hex\",\"00000022c4e0c07a\")"  ParamDataTypeStr=fixdt(1, 64, 40)  OutDataTypeStr=fixdt(1, 64, 40)  RndMeth=Convergent  SaturateOnIntegerOverflow=on  SampleTime=2e-08
  Goto2 : hdlmdlgenlib/Buffer
  Goto6 : hdlmdlgenlib/Buffer
  Ld : Constant  Value="fi(0,1,64,40,\"hex\",\"00000000725c3dee\")"  OutDataTypeStr=fixdt(1, 64, 40)  SampleTime=2e-08
  Product : Product  Inputs=**  OutDataTypeStr=fixdt(1, 64, 40)  RndMeth=Convergent  SaturateOnIntegerOverflow=on  SampleTime=2e-08
  Product1 : Product  Inputs=**  OutDataTypeStr=fixdt(1, 64, 40)  RndMeth=Convergent  SaturateOnIntegerOverflow=on  SampleTime=2e-08
  Reset_Integral : Switch  Criteria=u2 ~= 0  Threshold="fi(0,0,1,0,\"hex\",\"0\")"  OutDataTypeStr=fixdt(1, 64, 40)  RndMeth=Convergent  SampleTime=2e-08  InputSameDT=off
  Reset_Output : Switch  Criteria=u2 ~= 0  Threshold="fi(0,0,1,0,\"hex\",\"0\")"  OutDataTypeStr=fixdt(1, 64, 40)  RndMeth=Convergent  SampleTime=2e-08  InputSameDT=off
  Reset_Zero : Constant  Value="fi(0,1,64,40,\"hex\",\"0000000000000000\")"  OutDataTypeStr=fixdt(1, 64, 40)  SampleTime=2e-08
  Sum : Sum  Inputs=+-  OutDataTypeStr=fixdt(1, 64, 40)  AccumDataTypeStr=fixdt(1, 64, 40)  RndMeth=Convergent  SaturateOnIntegerOverflow=on  SampleTime=2e-08
  Sum1 : Sum  OutDataTypeStr=fixdt(1, 64, 40)  AccumDataTypeStr=fixdt(1, 64, 40)  RndMeth=Convergent  SaturateOnIntegerOverflow=on  SampleTime=2e-08
  crp_out_delay : Delay  DelayLength=1  InitialCondition=0  SampleTime=2e-08
  delayMatch : Delay  DelayLength=1  InitialCondition=0  SampleTime=2e-08
  delayMatch1 : Delay  DelayLength=1  InitialCondition=0  SampleTime=2e-08
  in1_repeat : RateTransition  Integrity=off  Deterministic=off  OutPortSampleTimeOpt=Multiple of input port sample time  OutPortSampleTimeMultiple=1/5000
  in2_repeat : RateTransition  Integrity=off  Deterministic=off  OutPortSampleTimeOpt=Multiple of input port sample time  OutPortSampleTimeMultiple=1/5000
  in3_repeat : RateTransition  Integrity=off  Deterministic=off  OutPortSampleTimeOpt=Multiple of input port sample time  OutPortSampleTimeMultiple=1/5000
  in6_repeat : RateTransition  Integrity=off  Deterministic=off  OutPortSampleTimeOpt=Multiple of input port sample time  OutPortSampleTimeMultiple=1/5000
  x_q_z : RateTransition  OutPortSampleTimeOpt=Multiple of input port sample time  OutPortSampleTimeMultiple=5000
  x_q_z_absorbed : Delay  DelayLength=0
  uq_raw : Outport  OutDataTypeStr=fixdt(1, 64, 40)  PortDimensions=1  SampleTime=2e-08
  wires:
  Ld/1 -> Product/2
  id/1 -> in6_repeat/1
  in6_repeat/1 -> Product/1
  Reset_Output/1 -> uq_raw/1
  Iq_ref/1 -> in2_repeat/1
  iq/1 -> in3_repeat/1
  Product/1 -> Add/1
  in2_repeat/1 -> Sum/1
  in3_repeat/1 -> Sum/2
  Constant/1 -> Add/2
  delayMatch1/1 -> Reset_Integral/2
  Sum/1 -> " "/1, "  "/1
  du_q_z/1 -> Goto2/1
  x_q_z_absorbed/1 -> in1_repeat/1
  "  "/1 -> Add1/1
  Add/1 -> Product1/1
  in1_repeat/1 -> Add2_stage2/1, Add1/2
  we/1 -> Product1/2
  " "/1 -> Add2_stage2/2
  Goto2/1 -> From6/1
  Add1/1 -> Sum1/1
  Product1/1 -> Sum1/2
  crp_out_delay/1 -> x_q_z/1
  Add2_stage2/1 -> delayMatch/1
  From6/1 -> Gain/1
  Reset_Zero/1 -> Reset_Integral/1, Reset_Output/1
  Sum1/1 -> Reset_Output/3
  PI_Reset_EN/1 -> delayMatch1/1, Reset_Output/2
  delayMatch/1 -> Add2_stage3/1
  Gain/1 -> Add2_stage3/2
  Add2_stage3/1 -> Reset_Integral/3
  Reset_Integral/1 -> Goto6/1
  Goto6/1 -> From2/1
  From2/1 -> crp_out_delay/1
  x_q_z/1 -> x_q_z_absorbed/1

== system gm_PMLSM_FOC_FixedPoint/FOC_DUT/FOC_DUT/Park ==
  A : Inport  OutDataTypeStr=fixdt(1,64,40,'DataTypeOverride', 'Off')  PortDimensions=1  SampleTime=0.0001
  B : Inport  Port=2  OutDataTypeStr=fixdt(1,64,40,'DataTypeOverride', 'Off')  PortDimensions=1  SampleTime=0.0001
  C : Inport  Port=3  OutDataTypeStr=fixdt(1,40,32,'DataTypeOverride', 'Off')  PortDimensions=1  SampleTime=0.0001
  Variant : Subsystem
  O1 : Outport  OutDataTypeStr=fixdt(1, 64, 40)  PortDimensions=1  SampleTime=0.0001
  O2 : Outport  Port=2  OutDataTypeStr=fixdt(1, 64, 40)  PortDimensions=1  SampleTime=0.0001
  wires:
  Variant/1(O1) -> O1/1
  A/1 -> Variant/1(A)
  B/1 -> Variant/2(B)
  C/1 -> Variant/3(C)
  Variant/2(O2) -> O2/1

== system gm_PMLSM_FOC_FixedPoint/FOC_DUT/FOC_DUT/SVPWMG ==
  Valpha : Inport  OutDataTypeStr=fixdt(1, 64, 40)  PortDimensions=1  SampleTime=2e-08
  Vbeta : Inport  Port=2  OutDataTypeStr=fixdt(1, 64, 40)  PortDimensions=1  SampleTime=2e-08
  Vdc_V : Inport  Port=3  OutDataTypeStr=fixdt(0, 32, 24)  PortDimensions=1  SampleTime=2e-08
  Duty Calculate : Subsystem
  Sector Caculate : Subsystem
  T1T2 Calculate : Subsystem
  XYZ Calculate : Subsystem
  duty_u_cmd : Outport  OutDataTypeStr=fixdt(1, 64, 40)  PortDimensions=1  SampleTime=2e-08
  duty_v_cmd : Outport  Port=2  OutDataTypeStr=fixdt(1, 64, 40)  PortDimensions=1  SampleTime=2e-08
  duty_w_cmd : Outport  Port=3  OutDataTypeStr=fixdt(1, 64, 40)  PortDimensions=1  SampleTime=2e-08
  wires:
  Valpha/1 -> XYZ Calculate/1(Ualpha), Sector Caculate/1(Ualpha)
  Duty Calculate/3(Duty_W) -> duty_w_cmd/1
  XYZ Calculate/2(Y) -> T1T2 Calculate/3(Y)
  Vbeta/1 -> Sector Caculate/2(Ubeta), XYZ Calculate/2(Ubeta)
  XYZ Calculate/3(Z) -> T1T2 Calculate/4(Z)
  Sector Caculate/1("N ") -> Duty Calculate/1(N), T1T2 Calculate/1(N)
  Vdc_V/1 -> XYZ Calculate/3(Udc)
  XYZ Calculate/1(X) -> T1T2 Calculate/2(X)
  T1T2 Calculate/1(T1) -> Duty Calculate/2(T1)
  T1T2 Calculate/2(T2) -> Duty Calculate/3(T2)
  Duty Calculate/1(Duty_U) -> duty_u_cmd/1
  Duty Calculate/2(Duty_V) -> duty_v_cmd/1

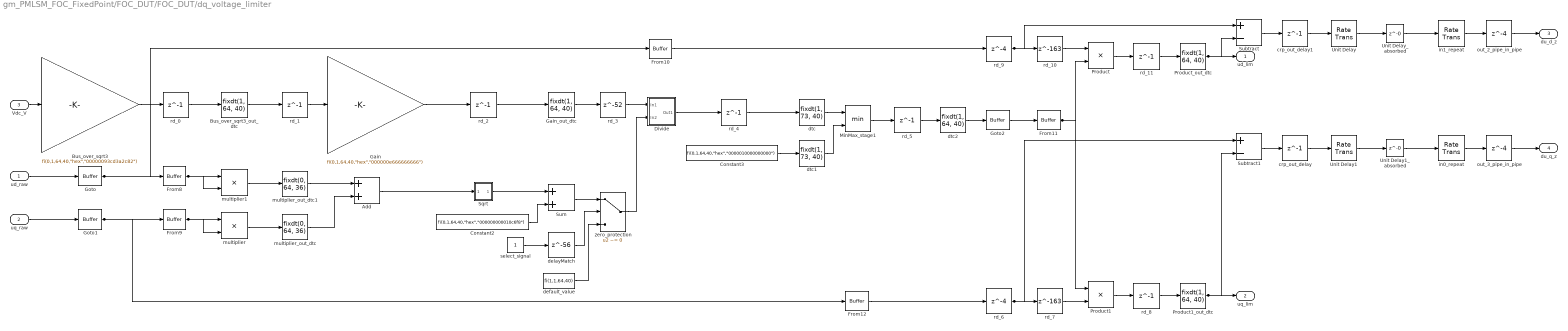
== system gm_PMLSM_FOC_FixedPoint/FOC_DUT/FOC_DUT/dq_voltage_limiter ==
  ud_raw : Inport  OutDataTypeStr=fixdt(1, 64, 40)  PortDimensions=1  SampleTime=2e-08
  uq_raw : Inport  Port=2  OutDataTypeStr=fixdt(1, 64, 40)  PortDimensions=1  SampleTime=2e-08
  Vdc_V : Inport  Port=3  OutDataTypeStr=fixdt(0, 32, 24)  PortDimensions=1  SampleTime=2e-08
  Add : Sum  OutDataTypeStr=fixdt(0, 64, 36)  AccumDataTypeStr=fixdt(0, 64, 36)  RndMeth=Convergent  SaturateOnIntegerOverflow=on  SampleTime=2e-08
  Bus_over_sqrt3 : Gain  Gain="fi(0,1,64,40,\"hex\",\"00000093cd3a2c82\")"  ParamDataTypeStr=fixdt(1, 64, 40)  OutDataTypeStr=fixdt(1, 96, 64)  SampleTime=2e-08
  Bus_over_sqrt3_out_dtc : DataTypeConversion  OutDataTypeStr=fixdt(1, 64, 40)  RndMeth=Convergent  SampleTime=2e-08
  Constant2 : Constant  Value="fi(0,1,64,40,\"hex\",\"000000000010c6f8\")"  OutDataTypeStr=fixdt(1, 64, 40)  SampleTime=2e-08
  Constant3 : Constant  Value="fi(0,1,64,40,\"hex\",\"0000010000000000\")"  OutDataTypeStr=fixdt(1, 64, 40)  SampleTime=2e-08
  Divide : Subsystem
  From{8..12} (5 alike) : hdlmdlgenlib/Buffer
  Gain : Gain  Gain="fi(0,1,64,40,\"hex\",\"000000e666666666\")"  ParamDataTypeStr=fixdt(1, 64, 40)  OutDataTypeStr=fixdt(1, 128, 80)  SampleTime=2e-08
  Gain_out_dtc : DataTypeConversion  OutDataTypeStr=fixdt(1, 64, 40)  RndMeth=Convergent  SampleTime=2e-08
  Goto : hdlmdlgenlib/Buffer
  Goto1 : hdlmdlgenlib/Buffer
  Goto2 : hdlmdlgenlib/Buffer
  MinMax_stage1 : MinMax  Inputs=2
  Product : Product  Inputs=**  OutDataTypeStr=fixdt(1, 128, 80)  SampleTime=2e-08
  Product1 : Product  Inputs=**  OutDataTypeStr=fixdt(1, 128, 80)  SampleTime=2e-08
  Product1_out_dtc : DataTypeConversion  OutDataTypeStr=fixdt(1, 64, 40)  RndMeth=Convergent  SampleTime=2e-08
  Product_out_dtc : DataTypeConversion  OutDataTypeStr=fixdt(1, 64, 40)  RndMeth=Convergent  SampleTime=2e-08
  Sqrt : Subsystem
  Subtract : Sum  Inputs=+-  OutDataTypeStr=fixdt(1, 64, 40)  AccumDataTypeStr=fixdt(1, 64, 40)  RndMeth=Convergent  SaturateOnIntegerOverflow=on  SampleTime=2e-08
  Subtract1 : Sum  Inputs=+-  OutDataTypeStr=fixdt(1, 64, 40)  AccumDataTypeStr=fixdt(1, 64, 40)  RndMeth=Convergent  SaturateOnIntegerOverflow=on  SampleTime=2e-08
  Sum : Sum  OutDataTypeStr=fixdt(1, 64, 40)  AccumDataTypeStr=fixdt(1, 64, 40)  RndMeth=Convergent  SaturateOnIntegerOverflow=on  SampleTime=2e-08
  Unit Delay : RateTransition  OutPortSampleTimeOpt=Multiple of input port sample time  OutPortSampleTimeMultiple=5000
  Unit Delay1 : RateTransition  OutPortSampleTimeOpt=Multiple of input port sample time  OutPortSampleTimeMultiple=5000
  Unit Delay1_absorbed : Delay  DelayLength=0
  Unit Delay_absorbed : Delay  DelayLength=0
  crp_out_delay : Delay  DelayLength=1  InitialCondition=0  SampleTime=2e-08
  crp_out_delay1 : Delay  DelayLength=1  InitialCondition=0  SampleTime=2e-08
  default_value : Constant  Value=fi(1,1,64,40)  OutDataTypeStr=fixdt(1, 64, 40)  SampleTime=2e-08
  delayMatch : Delay  DelayLength=56  InitialCondition=0  SampleTime=2e-08
  dtc : DataTypeConversion  OutDataTypeStr=fixdt(1, 73, 40)  RndMeth=Convergent  SampleTime=2e-08
  dtc1 : DataTypeConversion  OutDataTypeStr=fixdt(1, 73, 40)  RndMeth=Convergent  SampleTime=2e-08
  dtc2 : DataTypeConversion  OutDataTypeStr=fixdt(1, 64, 40)  RndMeth=Convergent  SampleTime=2e-08
  in0_repeat : RateTransition  Integrity=off  Deterministic=off  OutPortSampleTimeOpt=Multiple of input port sample time  OutPortSampleTimeMultiple=1/5000
  in1_repeat : RateTransition  Integrity=off  Deterministic=off  OutPortSampleTimeOpt=Multiple of input port sample time  OutPortSampleTimeMultiple=1/5000
  multiplier : Product  Inputs=**  OutDataTypeStr=fixdt(1, 128, 80)  SampleTime=2e-08
  multiplier1 : Product  Inputs=**  OutDataTypeStr=fixdt(1, 128, 80)  SampleTime=2e-08
  multiplier_out_dtc : DataTypeConversion  OutDataTypeStr=fixdt(0, 64, 36)  RndMeth=Convergent  SampleTime=2e-08
  multiplier_out_dtc1 : DataTypeConversion  OutDataTypeStr=fixdt(0, 64, 36)  RndMeth=Convergent  SampleTime=2e-08
  out_2_pipe_in_pipe : Delay  DelayLength=4  InitialCondition=0  SampleTime=2e-08
  out_3_pipe_in_pipe : Delay  DelayLength=4  InitialCondition=0  SampleTime=2e-08
  rd_{0..2,4..5,8,11} (7 alike) : Delay  DelayLength=1  InitialCondition=0  SampleTime=2e-08
  rd_10 : Delay  DelayLength=163  InitialCondition=0  SampleTime=2e-08
  rd_3 : Delay  DelayLength=52  InitialCondition=0  SampleTime=2e-08
  rd_6 : Delay  DelayLength=4  InitialCondition=0  SampleTime=2e-08
  rd_7 : Delay  DelayLength=163  InitialCondition=0  SampleTime=2e-08
  rd_9 : Delay  DelayLength=4  InitialCondition=0  SampleTime=2e-08
  select_signal : Constant  OutDataTypeStr=boolean  SampleTime=2e-08
  zero_protection : Switch  Criteria=u2 ~= 0  OutDataTypeStr=fixdt(1, 64, 40)  SampleTime=2e-08  SaturateOnIntegerOverflow=off  InputSameDT=off
  ud_lim : Outport  OutDataTypeStr=fixdt(1, 64, 40)  PortDimensions=1  SampleTime=2e-08
  uq_lim : Outport  Port=2  OutDataTypeStr=fixdt(1, 64, 40)  PortDimensions=1  SampleTime=2e-08
  du_d_z : Outport  Port=3  OutDataTypeStr=fixdt(1, 64, 40)  PortDimensions=1  SampleTime=2e-08
  du_q_z : Outport  Port=4  OutDataTypeStr=fixdt(1, 64, 40)  PortDimensions=1  SampleTime=2e-08
  wires:
  Unit Delay1/1 -> Unit Delay1_absorbed/1
  Vdc_V/1 -> Bus_over_sqrt3/1
  Unit Delay/1 -> Unit Delay_absorbed/1
  Add/1 -> Sqrt/1(In1)
  ud_raw/1 -> Goto/1
  Bus_over_sqrt3/1 -> rd_0/1
  Product_out_dtc/1 -> Subtract/2, ud_lim/1
  uq_raw/1 -> Goto1/1
  Goto/1 -> From10/1, From8/1
  From8/1 -> multiplier1/2, multiplier1/1
  rd_8/1 -> Product1_out_dtc/1
  Goto1/1 -> From12/1, From9/1
  Gain/1 -> rd_2/1
  rd_0/1 -> Bus_over_sqrt3_out_dtc/1
  From9/1 -> multiplier/2, multiplier/1
  Bus_over_sqrt3_out_dtc/1 -> rd_1/1
  rd_10/1 -> Product/1
  multiplier1/1 -> multiplier_out_dtc1/1
  rd_6/1 -> Subtract1/1, rd_7/1
  multiplier/1 -> multiplier_out_dtc/1
  rd_1/1 -> Gain/1
  multiplier_out_dtc1/1 -> Add/1
  multiplier_out_dtc/1 -> Add/2
  Constant2/1 -> Sum/2
  rd_2/1 -> Gain_out_dtc/1
  Sqrt/1(Out1) -> Sum/1
  Product1/1 -> rd_8/1
  select_signal/1 -> delayMatch/1
  Gain_out_dtc/1 -> rd_3/1
  Sum/1 -> zero_protection/1
  delayMatch/1 -> zero_protection/2
  Product/1 -> rd_11/1
  default_value/1 -> zero_protection/3
  rd_3/1 -> Divide/1(In1)
  Divide/1(Out1) -> rd_4/1
  zero_protection/1 -> Divide/2(In2)
  From10/1 -> rd_9/1
  rd_4/1 -> dtc/1
  Constant3/1 -> dtc1/1
  Unit Delay1_absorbed/1 -> in0_repeat/1
  dtc/1 -> MinMax_stage1/1
  Unit Delay_absorbed/1 -> in1_repeat/1
  dtc1/1 -> MinMax_stage1/2
  out_3_pipe_in_pipe/1 -> du_q_z/1
  MinMax_stage1/1 -> rd_5/1
  From12/1 -> rd_6/1
  From11/1 -> Product1/1, Product/2
  rd_5/1 -> dtc2/1
  dtc2/1 -> Goto2/1
  rd_9/1 -> Subtract/1, rd_10/1
  Goto2/1 -> From11/1
  rd_7/1 -> Product1/2
  rd_11/1 -> Product_out_dtc/1
  Product1_out_dtc/1 -> uq_lim/1, Subtract1/2
  crp_out_delay/1 -> Unit Delay1/1
  Subtract/1 -> crp_out_delay1/1
  Subtract1/1 -> crp_out_delay/1
  crp_out_delay1/1 -> Unit Delay/1
  in1_repeat/1 -> out_2_pipe_in_pipe/1
  in0_repeat/1 -> out_3_pipe_in_pipe/1
  out_2_pipe_in_pipe/1 -> du_d_z/1

== system gm_PMLSM_FOC_FixedPoint/FOC_DUT/FOC_DUT/InversePark/Variant ==
  A : Inport  OutDataTypeStr=fixdt(1, 64, 40)  PortDimensions=1  SampleTime=2e-08
  B : Inport  Port=2  OutDataTypeStr=fixdt(1, 64, 40)  PortDimensions=1  SampleTime=2e-08
  C : Inport  Port=3  OutDataTypeStr=fixdt(1, 40, 32)  PortDimensions=1  SampleTime=0.0001
  mcb : Subsystem
  O1 : Outport  OutDataTypeStr=fixdt(1, 64, 40)  PortDimensions=1  SampleTime=2e-08
  O2 : Outport  Port=2  OutDataTypeStr=fixdt(1, 64, 40)  PortDimensions=1  SampleTime=2e-08
  wires:
  A/1 -> mcb/1(A)
  B/1 -> mcb/2(B)
  C/1 -> mcb/3(C)
  mcb/1(O1) -> O1/1
  mcb/2(O2) -> O2/1

== system gm_PMLSM_FOC_FixedPoint/FOC_DUT/FOC_DUT/Park/Variant ==
  A : Inport  OutDataTypeStr=fixdt(1, 64, 40)  PortDimensions=1  SampleTime=0.0001
  B : Inport  Port=2  OutDataTypeStr=fixdt(1, 64, 40)  PortDimensions=1  SampleTime=0.0001
  C : Inport  Port=3  OutDataTypeStr=fixdt(1, 40, 32)  PortDimensions=1  SampleTime=0.0001
  mcb : Subsystem
  O1 : Outport  OutDataTypeStr=fixdt(1, 64, 40)  PortDimensions=1  SampleTime=0.0001
  O2 : Outport  Port=2  OutDataTypeStr=fixdt(1, 64, 40)  PortDimensions=1  SampleTime=0.0001
  wires:
  A/1 -> mcb/1(A)
  B/1 -> mcb/2(B)
  C/1 -> mcb/3(C)
  mcb/1(O1) -> O1/1
  mcb/2(O2) -> O2/1

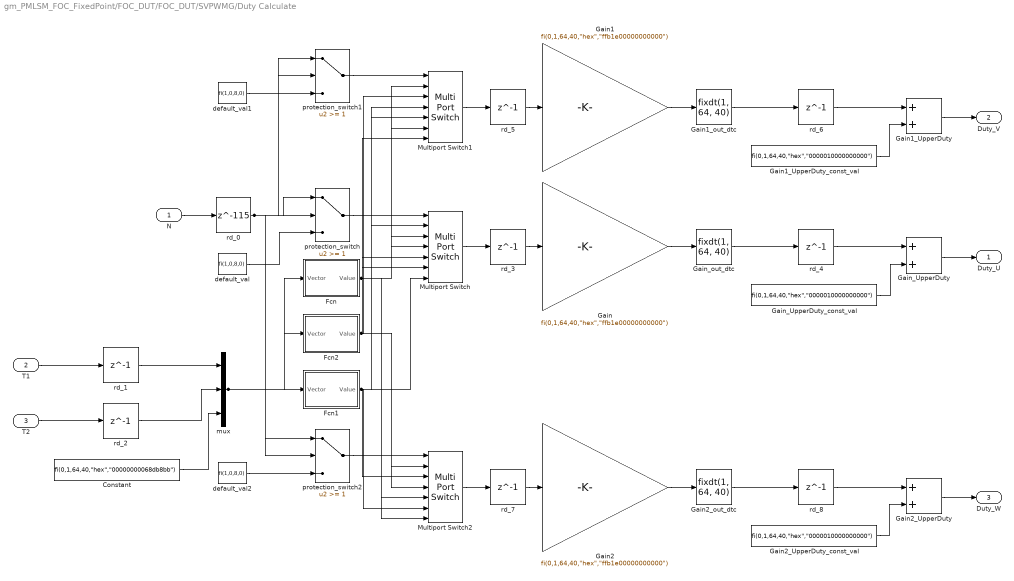
== system gm_PMLSM_FOC_FixedPoint/FOC_DUT/FOC_DUT/SVPWMG/Duty Calculate ==
  N : Inport  OutDataTypeStr=uint8  PortDimensions=1  SampleTime=2e-08
  T1 : Inport  Port=2  OutDataTypeStr=fixdt(1, 64, 40)  PortDimensions=1  SampleTime=2e-08
  T2 : Inport  Port=3  OutDataTypeStr=fixdt(1, 64, 40)  PortDimensions=1  SampleTime=2e-08
  Constant : Constant  Value="fi(0,1,64,40,\"hex\",\"00000000068db8bb\")"  OutDataTypeStr=fixdt(1, 64, 40)  SampleTime=2e-08
  Fcn : Subsystem
  Fcn1 : Subsystem
  Fcn2 : Subsystem
  Gain : Gain  Gain="fi(0,1,64,40,\"hex\",\"ffb1e00000000000\")"  ParamDataTypeStr=fixdt(1, 64, 40)  OutDataTypeStr=fixdt(1, 128, 80)  SampleTime=2e-08
  Gain1 : Gain  Gain="fi(0,1,64,40,\"hex\",\"ffb1e00000000000\")"  ParamDataTypeStr=fixdt(1, 64, 40)  OutDataTypeStr=fixdt(1, 128, 80)  SampleTime=2e-08
  Gain1_UpperDuty : Sum  OutDataTypeStr=fixdt(1, 64, 40)  AccumDataTypeStr=fixdt(1, 64, 40)  RndMeth=Nearest  SaturateOnIntegerOverflow=on  SampleTime=2e-08
  Gain1_UpperDuty_const_val : Constant  Value="fi(0,1,64,40,\"hex\",\"0000010000000000\")"  VectorParams1D=off  OutDataTypeStr=fixdt(1, 64, 40)  SampleTime=2e-08
  Gain1_out_dtc : DataTypeConversion  OutDataTypeStr=fixdt(1, 64, 40)  RndMeth=Convergent  SampleTime=2e-08
  Gain2 : Gain  Gain="fi(0,1,64,40,\"hex\",\"ffb1e00000000000\")"  ParamDataTypeStr=fixdt(1, 64, 40)  OutDataTypeStr=fixdt(1, 128, 80)  SampleTime=2e-08
  Gain2_UpperDuty : Sum  OutDataTypeStr=fixdt(1, 64, 40)  AccumDataTypeStr=fixdt(1, 64, 40)  RndMeth=Nearest  SaturateOnIntegerOverflow=on  SampleTime=2e-08
  Gain2_UpperDuty_const_val : Constant  Value="fi(0,1,64,40,\"hex\",\"0000010000000000\")"  VectorParams1D=off  OutDataTypeStr=fixdt(1, 64, 40)  SampleTime=2e-08
  Gain2_out_dtc : DataTypeConversion  OutDataTypeStr=fixdt(1, 64, 40)  RndMeth=Convergent  SampleTime=2e-08
  Gain_UpperDuty : Sum  OutDataTypeStr=fixdt(1, 64, 40)  AccumDataTypeStr=fixdt(1, 64, 40)  RndMeth=Nearest  SaturateOnIntegerOverflow=on  SampleTime=2e-08
  Gain_UpperDuty_const_val : Constant  Value="fi(0,1,64,40,\"hex\",\"0000010000000000\")"  VectorParams1D=off  OutDataTypeStr=fixdt(1, 64, 40)  SampleTime=2e-08
  Gain_out_dtc : DataTypeConversion  OutDataTypeStr=fixdt(1, 64, 40)  RndMeth=Convergent  SampleTime=2e-08
  Multiport Switch : MultiPortSwitch  Inputs=6  DiagnosticForDefault=None  OutDataTypeStr=fixdt(1, 64, 40)  RndMeth=Convergent  SampleTime=2e-08  InputSameDT=off
  Multiport Switch1 : MultiPortSwitch  Inputs=6  DiagnosticForDefault=None  OutDataTypeStr=fixdt(1, 64, 40)  RndMeth=Convergent  SampleTime=2e-08  InputSameDT=off
  Multiport Switch2 : MultiPortSwitch  Inputs=6  DiagnosticForDefault=None  OutDataTypeStr=fixdt(1, 64, 40)  RndMeth=Convergent  SampleTime=2e-08  InputSameDT=off
  default_val : Constant  Value=fi(1,0,8,0)  OutDataTypeStr=uint8  SampleTime=2e-08
  default_val1 : Constant  Value=fi(1,0,8,0)  OutDataTypeStr=uint8  SampleTime=2e-08
  default_val2 : Constant  Value=fi(1,0,8,0)  OutDataTypeStr=uint8  SampleTime=2e-08
  mux : Mux  Inputs=3
  protection_switch : Switch  Threshold=1  OutDataTypeStr=uint8  SampleTime=2e-08  SaturateOnIntegerOverflow=off  InputSameDT=off
  protection_switch1 : Switch  Threshold=1  OutDataTypeStr=uint8  SampleTime=2e-08  SaturateOnIntegerOverflow=off  InputSameDT=off
  protection_switch2 : Switch  Threshold=1  OutDataTypeStr=uint8  SampleTime=2e-08  SaturateOnIntegerOverflow=off  InputSameDT=off
  rd_0 : Delay  DelayLength=115  InitialCondition=0  SampleTime=2e-08
  rd_{1..8} (8 alike) : Delay  DelayLength=1  InitialCondition=0  SampleTime=2e-08
  Duty_U : Outport  OutDataTypeStr=fixdt(1, 64, 40)  PortDimensions=1  SampleTime=2e-08
  Duty_V : Outport  Port=2  OutDataTypeStr=fixdt(1, 64, 40)  PortDimensions=1  SampleTime=2e-08
  Duty_W : Outport  Port=3  OutDataTypeStr=fixdt(1, 64, 40)  PortDimensions=1  SampleTime=2e-08
  wires:
  Gain1_UpperDuty_const_val/1 -> Gain1_UpperDuty/2
  T1/1 -> rd_1/1
  rd_8/1 -> Gain2_UpperDuty/1
  T2/1 -> rd_2/1
  protection_switch1/1 -> Multiport Switch1/1
  Constant/1 -> mux/3
  rd_7/1 -> Gain2/1
  N/1 -> rd_0/1
  rd_1/1 -> mux/1
  Multiport Switch/1 -> rd_3/1
  rd_2/1 -> mux/2
  default_val1/1 -> protection_switch1/3
  rd_0/1 -> protection_switch1/1, protection_switch2/1, protection_switch1/2, protection_switch/1, protection_switch2/2, protection_switch/2
  default_val/1 -> protection_switch/3
  Gain1_out_dtc/1 -> rd_6/1
  mux/1 -> Fcn/1(Vector), Fcn1/1(Vector), Fcn2/1(Vector)
  Multiport Switch1/1 -> rd_5/1
  default_val2/1 -> protection_switch2/3
  protection_switch/1 -> Multiport Switch/1
  Fcn/1(Value) -> Multiport Switch2/7, Multiport Switch2/5, Multiport Switch1/6, Multiport Switch/4, Multiport Switch/3, Multiport Switch1/2
  Fcn2/1(Value) -> Multiport Switch2/2, Multiport Switch1/7, Multiport Switch/6, Multiport Switch/5, Multiport Switch1/3, Multiport Switch2/4
  Fcn1/1(Value) -> Multiport Switch2/3, Multiport Switch1/4, Multiport Switch/7, Multiport Switch/2, Multiport Switch1/5, Multiport Switch2/6
  protection_switch2/1 -> Multiport Switch2/1
  Gain/1 -> Gain_out_dtc/1
  Multiport Switch2/1 -> rd_7/1
  Gain1_UpperDuty/1 -> Duty_V/1
  rd_5/1 -> Gain1/1
  rd_3/1 -> Gain/1
  Gain1/1 -> Gain1_out_dtc/1
  Gain2_out_dtc/1 -> rd_8/1
  Gain2/1 -> Gain2_out_dtc/1
  Gain_out_dtc/1 -> rd_4/1
  Gain2_UpperDuty/1 -> Duty_W/1
  rd_6/1 -> Gain1_UpperDuty/1
  Gain_UpperDuty/1 -> Duty_U/1
  rd_4/1 -> Gain_UpperDuty/1
  Gain_UpperDuty_const_val/1 -> Gain_UpperDuty/2
  Gain2_UpperDuty_const_val/1 -> Gain2_UpperDuty/2

== system gm_PMLSM_FOC_FixedPoint/FOC_DUT/FOC_DUT/SVPWMG/Sector Caculate ==
  Ualpha : Inport  OutDataTypeStr=fixdt(1, 64, 40)  PortDimensions=1  SampleTime=2e-08
  Ubeta : Inport  Port=2  OutDataTypeStr=fixdt(1, 64, 40)  PortDimensions=1  SampleTime=2e-08
  B0 : Subsystem
  B1 : Subsystem
  B2 : Subsystem
  Constant : Constant  OutDataTypeStr=uint8  SampleTime=2e-08
  Constant1 : Constant  Value=0  OutDataTypeStr=uint8  SampleTime=2e-08
  N : Subsystem
  Switch : Switch  Criteria=u2 > Threshold  Threshold="fi(0,1,64,40,\"hex\",\"0000000000000000\")"  OutDataTypeStr=uint8  RndMeth=Convergent  SampleTime=2e-08  InputSameDT=off
  Switch1 : Switch  Threshold="fi(0,1,64,40,\"hex\",\"0000000000000000\")"  OutDataTypeStr=uint8  RndMeth=Convergent  SampleTime=2e-08  InputSameDT=off
  Switch2 : Switch  Criteria=u2 > Threshold  Threshold="fi(0,1,64,40,\"hex\",\"0000000000000000\")"  OutDataTypeStr=uint8  RndMeth=Convergent  SampleTime=2e-08  InputSameDT=off
  mux : Mux  Inputs=2
  mux1 : Mux  Inputs=3
  rd_0 : Delay  DelayLength=1  InitialCondition=0  SampleTime=2e-08
  "N " : Outport  OutDataTypeStr=uint8  PortDimensions=1  SampleTime=2e-08  VectorParamsAs1DForOutWhenUnconnected=off
  wires:
  Ualpha/1 -> mux/1
  Ubeta/1 -> mux/2
  Constant/1 -> Switch2/1, Switch1/1, Switch/1
  B2/1(Value) -> Switch2/2
  N/1(Value) -> "N "/1
  mux/1 -> B0/1(Vector), B1/1(Vector), B2/1(Vector)
  B0/1(Value) -> Switch/2
  Constant1/1 -> Switch2/3, Switch1/3, Switch/3
  B1/1(Value) -> Switch1/2
  Switch1/1 -> mux1/2
  Switch/1 -> rd_0/1
  Switch2/1 -> mux1/3
  rd_0/1 -> mux1/1
  mux1/1 -> N/1(Vector)

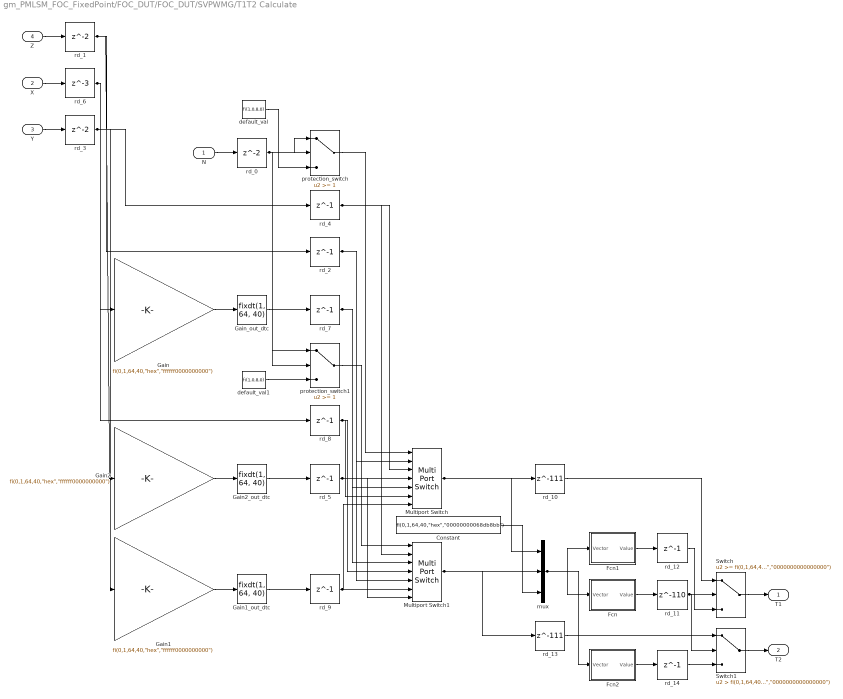
== system gm_PMLSM_FOC_FixedPoint/FOC_DUT/FOC_DUT/SVPWMG/T1T2 Calculate ==
  N : Inport  OutDataTypeStr=uint8  PortDimensions=1  SampleTime=2e-08
  X : Inport  Port=2  OutDataTypeStr=fixdt(1, 64, 40)  PortDimensions=1  SampleTime=2e-08
  Y : Inport  Port=3  OutDataTypeStr=fixdt(1, 64, 40)  PortDimensions=1  SampleTime=2e-08
  Z : Inport  Port=4  OutDataTypeStr=fixdt(1, 64, 40)  PortDimensions=1  SampleTime=2e-08
  Constant : Constant  Value="fi(0,1,64,40,\"hex\",\"00000000068db8bb\")"  OutDataTypeStr=fixdt(1, 64, 40)  SampleTime=2e-08
  Fcn : Subsystem
  Fcn1 : Subsystem
  Fcn2 : Subsystem
  Gain : Gain  Gain="fi(0,1,64,40,\"hex\",\"ffffff0000000000\")"  ParamDataTypeStr=fixdt(1, 64, 40)  OutDataTypeStr=fixdt(1, 128, 80)  SampleTime=2e-08
  Gain1 : Gain  Gain="fi(0,1,64,40,\"hex\",\"ffffff0000000000\")"  ParamDataTypeStr=fixdt(1, 64, 40)  OutDataTypeStr=fixdt(1, 128, 80)  SampleTime=2e-08
  Gain1_out_dtc : DataTypeConversion  OutDataTypeStr=fixdt(1, 64, 40)  RndMeth=Convergent  SampleTime=2e-08
  Gain2 : Gain  Gain="fi(0,1,64,40,\"hex\",\"ffffff0000000000\")"  ParamDataTypeStr=fixdt(1, 64, 40)  OutDataTypeStr=fixdt(1, 128, 80)  SampleTime=2e-08
  Gain2_out_dtc : DataTypeConversion  OutDataTypeStr=fixdt(1, 64, 40)  RndMeth=Convergent  SampleTime=2e-08
  Gain_out_dtc : DataTypeConversion  OutDataTypeStr=fixdt(1, 64, 40)  RndMeth=Convergent  SampleTime=2e-08
  Multiport Switch : MultiPortSwitch  Inputs=6  DiagnosticForDefault=None  OutDataTypeStr=fixdt(1, 64, 40)  RndMeth=Convergent  SampleTime=2e-08  InputSameDT=off
  Multiport Switch1 : MultiPortSwitch  Inputs=6  DiagnosticForDefault=None  OutDataTypeStr=fixdt(1, 64, 40)  RndMeth=Convergent  SampleTime=2e-08  InputSameDT=off
  Switch : Switch  Threshold="fi(0,1,64,40,\"hex\",\"0000000000000000\")"  OutDataTypeStr=fixdt(1, 64, 40)  RndMeth=Convergent  SampleTime=2e-08  InputSameDT=off
  Switch1 : Switch  Criteria=u2 > Threshold  Threshold="fi(0,1,64,40,\"hex\",\"0000000000000000\")"  OutDataTypeStr=fixdt(1, 64, 40)  RndMeth=Convergent  SampleTime=2e-08  InputSameDT=off
  default_val : Constant  Value=fi(1,0,8,0)  OutDataTypeStr=uint8  SampleTime=2e-08
  default_val1 : Constant  Value=fi(1,0,8,0)  OutDataTypeStr=uint8  SampleTime=2e-08
  mux : Mux  Inputs=3
  protection_switch : Switch  Threshold=1  OutDataTypeStr=uint8  SampleTime=2e-08  SaturateOnIntegerOverflow=off  InputSameDT=off
  protection_switch1 : Switch  Threshold=1  OutDataTypeStr=uint8  SampleTime=2e-08  SaturateOnIntegerOverflow=off  InputSameDT=off
  rd_0 : Delay  InitialCondition=0  SampleTime=2e-08
  rd_1 : Delay  InitialCondition=0  SampleTime=2e-08
  rd_10 : Delay  DelayLength=111  InitialCondition=0  SampleTime=2e-08
  rd_11 : Delay  DelayLength=110  InitialCondition=0  SampleTime=2e-08
  rd_{2,4..5,7..9,12,14} (8 alike) : Delay  DelayLength=1  InitialCondition=0  SampleTime=2e-08
  rd_13 : Delay  DelayLength=111  InitialCondition=0  SampleTime=2e-08
  rd_3 : Delay  InitialCondition=0  SampleTime=2e-08
  rd_6 : Delay  DelayLength=3  InitialCondition=0  SampleTime=2e-08
  T1 : Outport  OutDataTypeStr=fixdt(1, 64, 40)  PortDimensions=1  SampleTime=2e-08  VectorParamsAs1DForOutWhenUnconnected=off
  T2 : Outport  Port=2  OutDataTypeStr=fixdt(1, 64, 40)  PortDimensions=1  SampleTime=2e-08  VectorParamsAs1DForOutWhenUnconnected=off
  wires:
  rd_13/1 -> Switch1/1
  Z/1 -> rd_1/1
  X/1 -> rd_6/1
  rd_6/1 -> rd_8/1, Gain/1
  Switch1/1 -> T2/1
  Y/1 -> rd_3/1
  rd_12/1 -> Switch/3
  Gain/1 -> Gain_out_dtc/1
  rd_1/1 -> Gain2/1, rd_2/1
  rd_3/1 -> rd_4/1, Gain1/1
  Gain2/1 -> Gain2_out_dtc/1
  N/1 -> rd_0/1
  rd_10/1 -> Switch/1
  Gain1/1 -> Gain1_out_dtc/1
  default_val/1 -> protection_switch/3
  rd_0/1 -> protection_switch1/2, protection_switch/1, protection_switch1/1, protection_switch/2
  Gain_out_dtc/1 -> rd_7/1
  default_val1/1 -> protection_switch1/3
  Fcn2/1(Value) -> rd_14/1
  Gain2_out_dtc/1 -> rd_5/1
  Gain1_out_dtc/1 -> rd_9/1
  protection_switch/1 -> Multiport Switch/1
  rd_4/1 -> Multiport Switch1/2, Multiport Switch/3
  rd_2/1 -> Multiport Switch1/5, Multiport Switch/2
  rd_7/1 -> Multiport Switch/5, Multiport Switch1/3
  protection_switch1/1 -> Multiport Switch1/1
  rd_8/1 -> Multiport Switch1/4, Multiport Switch/6
  Fcn/1(Value) -> rd_11/1
  rd_5/1 -> Multiport Switch/4, Multiport Switch1/7
  rd_9/1 -> Multiport Switch1/6, Multiport Switch/7
  Multiport Switch/1 -> mux/1, rd_10/1
  Constant/1 -> mux/3
  Multiport Switch1/1 -> mux/2, rd_13/1
  mux/1 -> Fcn1/1(Vector), Fcn2/1(Vector), Fcn/1(Vector)
  Fcn1/1(Value) -> rd_12/1
  rd_11/1 -> Switch/2, Switch1/2
  rd_14/1 -> Switch1/3
  Switch/1 -> T1/1
